simulink model "bmsreq_can_pack"  (R2026b)
settings: Solver=VariableStepAuto
undefined symbols (not defined in the file or in its folder): Ts
libraries: simulink x1, svdutilitieslib x1
settings Model: Creator=aomar  LastModifiedBy=aomar

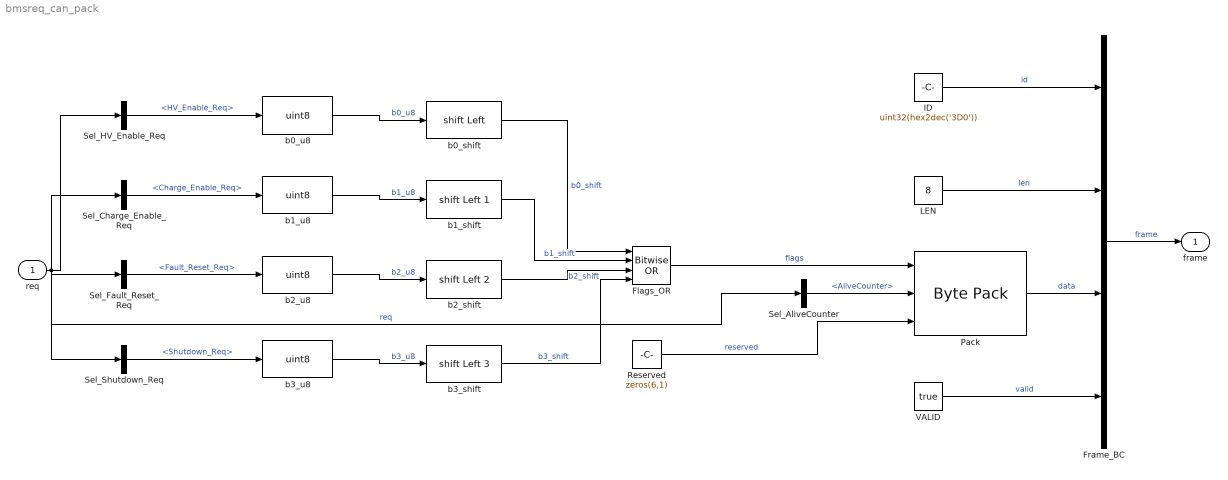
== system bmsreq_can_pack ==
  req : Inport  OutDataTypeStr=Bus: Bus_BmsReq  SampleTime=Ts.can_slow
  Flags_OR : simulink/Logic and Bit Operations/Bitwise Operator  logicop=OR  UseBitMask=off  NumInputPorts=4  BitMask=bin2dec('11011001')  BitMaskRealWorld=Stored Integer
  Frame_BC : BusCreator  Inputs=4  OutDataTypeStr=Bus: Bus_CanFrame8  NonVirtualBus=on
      settings: InheritFromInputs=off
  ID : Constant  Value=uint32(hex2dec('3D0'))  OutDataTypeStr=uint32  SampleTime=Ts.can_slow
  LEN : Constant  Value=8  OutDataTypeStr=uint8  SampleTime=Ts.can_slow
  Pack : svdutilitieslib/Byte Pack  maskPackedDataType=uint8  datatypes={'uint8','uint8','uint8'}  byteAlign=1  blockPlatform=arduinoert
      settings: LibrarySourceBlock=mcblib/Signal Management/Byte Pack
  Reserved : Constant  Value=zeros(6,1)  OutDataTypeStr=uint8  SampleTime=Ts.can_slow
  Sel_AliveCounter : BusSelector  OutputSignals=AliveCounter
  Sel_Charge_Enable_Req : BusSelector  OutputSignals=Charge_Enable_Req
  Sel_Fault_Reset_Req : BusSelector  OutputSignals=Fault_Reset_Req
  Sel_HV_Enable_Req : BusSelector  OutputSignals=HV_Enable_Req
  Sel_Shutdown_Req : BusSelector  OutputSignals=Shutdown_Req
  VALID : Constant  Value=true  OutDataTypeStr=boolean  SampleTime=Ts.can_slow
  b0_shift : ArithShift  BitShiftDirection=Left
  b0_u8 : DataTypeConversion  OutDataTypeStr=uint8  RndMeth=Nearest
  b1_shift : ArithShift  BitShiftNumber=1  BitShiftDirection=Left
  b1_u8 : DataTypeConversion  OutDataTypeStr=uint8  RndMeth=Nearest
  b2_shift : ArithShift  BitShiftNumber=2  BitShiftDirection=Left
  b2_u8 : DataTypeConversion  OutDataTypeStr=uint8  RndMeth=Nearest
  b3_shift : ArithShift  BitShiftNumber=3  BitShiftDirection=Left
  b3_u8 : DataTypeConversion  OutDataTypeStr=uint8  RndMeth=Nearest
  frame : Outport  OutDataTypeStr=Bus: Bus_CanFrame8
  wires:
  req/1 -> Sel_HV_Enable_Req/1, Sel_Shutdown_Req/1, Sel_Charge_Enable_Req/1, Sel_AliveCounter/1, Sel_Fault_Reset_Req/1  "req"
  Sel_HV_Enable_Req/1 -> b0_u8/1  "<HV_Enable_Req>"
  Sel_Charge_Enable_Req/1 -> b1_u8/1  "<Charge_Enable_Req>"
  Sel_Fault_Reset_Req/1 -> b2_u8/1  "<Fault_Reset_Req>"
  Sel_Shutdown_Req/1 -> b3_u8/1  "<Shutdown_Req>"
  b0_u8/1 -> b0_shift/1  "b0_u8"
  b1_u8/1 -> b1_shift/1  "b1_u8"
  b2_u8/1 -> b2_shift/1  "b2_u8"
  b3_u8/1 -> b3_shift/1  "b3_u8"
  b0_shift/1 -> Flags_OR/1  "b0_shift"
  b1_shift/1 -> Flags_OR/2  "b1_shift"
  b2_shift/1 -> Flags_OR/3  "b2_shift"
  b3_shift/1 -> Flags_OR/4  "b3_shift"
  Reserved/1 -> Pack/3  "reserved"
  Flags_OR/1 -> Pack/1  "flags"
  Sel_AliveCounter/1 -> Pack/2  "<AliveCounter>"
  ID/1 -> Frame_BC/1  "id"
  LEN/1 -> Frame_BC/2  "len"
  VALID/1 -> Frame_BC/4  "valid"
  Pack/1 -> Frame_BC/3  "data"
  Frame_BC/1 -> frame/1  "frame"
